simulink model "TP7_commande_automat_capot"  (R2022b)
settings: Solver=VariableStepAuto  StartTime=0.0  StopTime=inf  RelTol=1e-3
settings Model: Creator=HP  LastModifiedBy=HP

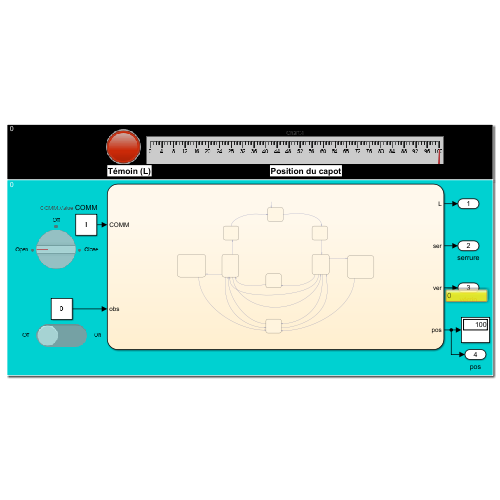
[thumbnail: Simulink's stored preview of the top-level diagram]
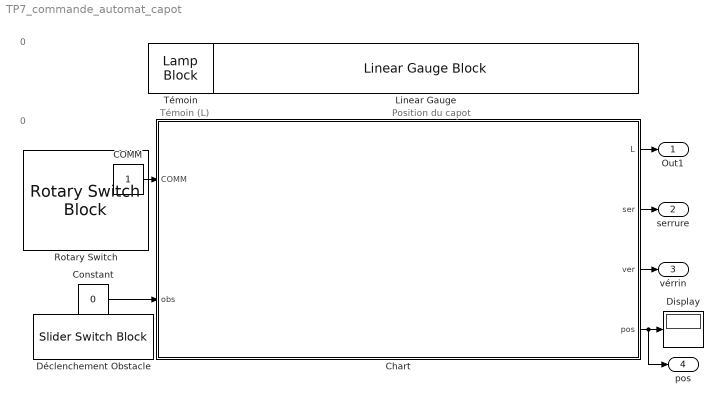
== system TP7_commande_automat_capot ==
  note: Position du capot
  note: Témoin (L)
  note: 0
  note: 0
  COMM : Constant
  Chart : Stateflow chart  TreatAsAtomicUnit=on
  Constant : Constant  Value=0
  Display : Display
  Déclenchement Obstacle : SliderSwitchBlock  LabelPosition=Hide
      settings: Values={{'Off', 'On'}, [0 1]}
  Linear Gauge : LinearGaugeBlock
  Rotary Switch : RotarySwitchBlock
      settings: Values={{'Open', 'Off', 'Close'}, [1 0 2]}
  Témoin : LampBlock  LabelPosition=Hide
  Out1 : Outport
  serrure : Outport  Port=2
  vérrin : Outport  Port=3
  pos : Outport  Port=4
  wires:
  Chart/3(ver) -> vérrin/1
  Chart/1(L) -> Out1/1
  COMM/1 -> Chart/1(COMM)
  Chart/2(ser) -> serrure/1
  Chart/4(pos) -> pos/1, Display/1
  Constant/1 -> Chart/2(obs)

== stateflow chart TP7_commande_automat_capot/Chart ==
  settings: updateMethod=DISCRETE  sampleTime=0.5/3
  state repos
    entry:
    L=0;
    ser=0;
    ver=0;
  state verrouillage
    entry:
    L=1;
    ser=0;
    ver=0;
  state deverrouillage
    entry:
    L=1;
    ser=1;
    ver=0;
  state recul_haut
    entry:
    L=1;
    ser=1;
    ver=1;
    cible = min(pos + 10, 100)
    during:
    pos = pos + 1;
  state fermeture
    entry:
    L=1;
    ser=1;
    ver = -1;
    during:
    pos = pos - 1;
  state ouverture
    entry:
    L=1;
    ser=1;
    ver=1;
    during:
    pos = pos + 1;
  state recul_bas
    entry:
    L=1;
    ser=1;
    ver = -1;
    cible = max(pos - 10, 0)
    during:
    pos = pos - 1;
  state ouvert
    entry:
    L=1;
    ser=1;
    ver=0;
  state arret
    entry:
    L=1;
    ser=1;
    ver=0;
  (default) -> repos
  repos -> deverrouillage : [COMM == 1]
  verrouillage -> repos : [after(1, sec)]
  fermeture -> verrouillage [order 2] : [pos <= 0]
  deverrouillage -> ouverture : [after(1, sec)]
  ouverture -> recul_bas [order 2] : [obs == 1]
  fermeture -> recul_haut [order 3] : [obs == 1]
  ouverture -> arret [order 4] : [COMM == 0]
  arret -> ouverture [order 1] : [COMM == 1 && obs == 0]
  ouverture -> fermeture [order 3] : [obs == 0 && COMM == 2]
  fermeture -> ouverture [order 1] : [obs == 0 && COMM == 1]
  ouverture -> ouvert [order 1] : [pos >= 100]
  recul_haut -> arret : [pos >= cible]
  fermeture -> arret [order 4] : [COMM==0]
  arret -> fermeture [order 2] : [obs == 0 && COMM == 2]
  ouvert -> fermeture : [COMM == 2]
  recul_bas -> arret : [pos <= cible]
  data: COMM input; L output; ser output; ver output; pos output double size=1 =0; obs input double size=1; cible local
